simulink model "RCAM_PID_takeoff_lamding_20261013_step02"  (R2024b)
settings: Solver=VariableStepAuto  StartTime=0.0  StopTime=4200  MaxStep=0.01  RelTol=1e-3
undefined symbols (not defined in the file or in its folder): RCAM_dynamics_fcn20261013_step02_brake, RCAM_monitor_20261013_step02
libraries: simulink x28, slpidlib x9, simulink_extras x2
(part 2 of 2)

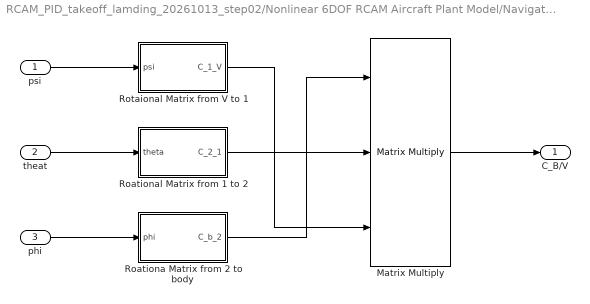
== system RCAM_PID_takeoff_lamding_20261013_step02/Nonlinear 6DOF RCAM Aircraft Plant Model/Navigational BLOCK/Navigational Equation ==
  psi : Inport
  theat : Inport  Port=2
  phi : Inport  Port=3
  Matrix Multiply : Product  Inputs=3  Multiplication=Matrix(*)
  Roationa Matrix from 2 to body : MATLAB Function  TreatAsAtomicUnit=on
  Roational Matrix from 1 to 2 : MATLAB Function  TreatAsAtomicUnit=on
  Rotaional Matrix from V to 1 : MATLAB Function  TreatAsAtomicUnit=on
  C_B/V : Outport
  wires:
  psi/1 -> Rotaional Matrix from V to 1/1(psi)
  theat/1 -> Roational Matrix from 1 to 2/1(theta)
  phi/1 -> Roationa Matrix from 2 to body/1(phi)
  Roationa Matrix from 2 to body/1(C_b_2) -> Matrix Multiply/1
  Roational Matrix from 1 to 2/1(C_2_1) -> Matrix Multiply/2
  Rotaional Matrix from V to 1/1(C_1_V) -> Matrix Multiply/3
  Matrix Multiply/1 -> C_B/V/1

== matlab function RCAM_PID_takeoff_lamding_20261013_step02/Nonlinear 6DOF RCAM Aircraft Plant Model/Navigational BLOCK/Navigational Equation/Roational Matrix from 1 to 2 ==
  data: theta input; C_2_1 output
function C_2_1 = fcn(theta)

% Roational Matrix From the 1 frame to 2 frame

C_2_1=[cos(theta) 0 -sin(theta); 0 1 0; sin(theta) 0 cos(theta)];

end

== matlab function RCAM_PID_takeoff_lamding_20261013_step02/Nonlinear 6DOF RCAM Aircraft Plant Model/Navigational BLOCK/Navigational Equation/Rotaional Matrix from V to 1 ==
  data: psi input; C_1_V output
function C_1_V = fcn(psi)

% Calculating the Rotaional Matrix  from the NED to 1 frame

C_1_V=[cos(psi) sin(psi) 0; -sin(psi) cos(psi) 0; 0 0 1];

end

== matlab function RCAM_PID_takeoff_lamding_20261013_step02/Nonlinear 6DOF RCAM Aircraft Plant Model/Navigational BLOCK/Navigational Equation/Roationa Matrix from 2 to body ==
  data: phi input; C_b_2 output
function C_b_2 = fcn(phi)

% Roational Matrix from the 2 frame to body frame
C_b_2=[1 0 0; 0 cos(phi) sin(phi); 0 -sin(phi) cos(phi)];
end
